simulink model "tb_q_current_control_basics"  (R2025b)
settings: Solver=VariableStepAuto  StartTime=0.0  StopTime=0.02  RelTol=1e-3
settings Model: Creator=semih  LastModifiedBy=semih

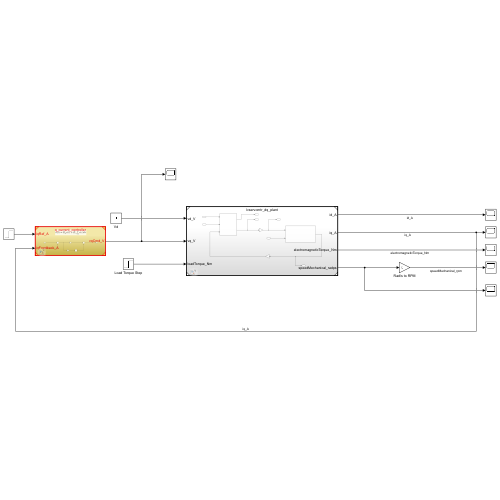
[thumbnail: Simulink's stored preview of the top-level diagram]
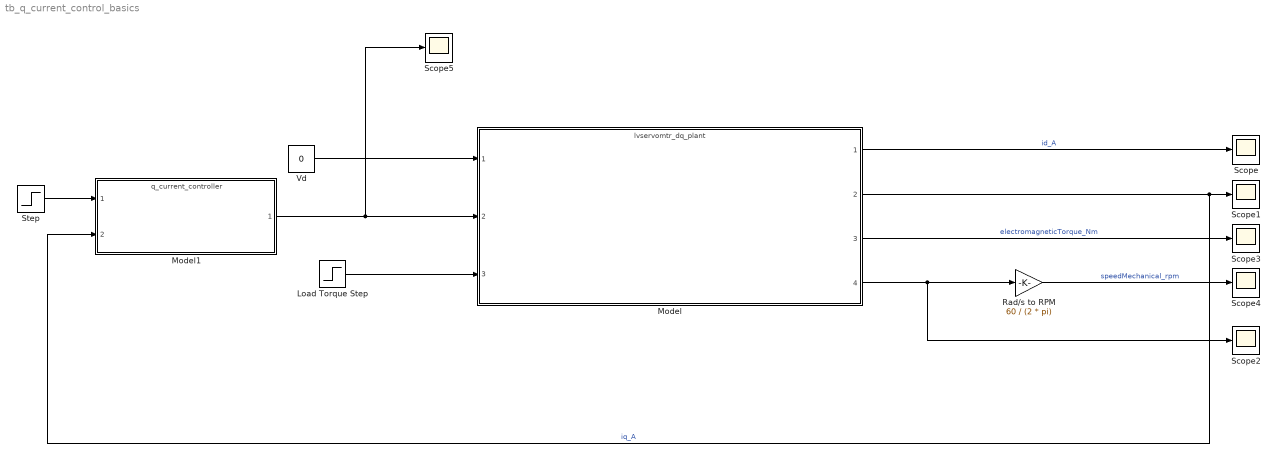
== system tb_q_current_control_basics ==
  Load Torque Step : Step  Time=0.030  After=0  SampleTime=0
  Model : ModelReference  ModelNameDialog=lvservomtr_dq_plant  SimulationMode=Normal  ModelReferenceVersion=1.7
  Model1 : ModelReference  ModelNameDialog=q_current_controller.slx  SimulationMode=Normal  ModelReferenceVersion=1.3
  Rad/s to RPM : Gain  Gain=60 / (2 * pi)
  Scope{,1..5} (6 alike) : Scope
      Scope settings: ActiveDisplayYMinimum=-0.42366511792142403  ActiveDisplayYMaximum=1.8876545573518515
      Scope1 settings: ActiveDisplayYMinimum=-0.63597233219420146  ActiveDisplayYMaximum=2.1211566623596005
      Scope2 settings: ActiveDisplayYMinimum=-14.648422716149396  ActiveDisplayYMaximum=131.83580444534459  DataLoggingVariableName=ScopeData2
      Scope3 settings: ActiveDisplayYMinimum=-0.077109095292808  ActiveDisplayYMaximum=0.69398185763527209  DataLoggingVariableName=ScopeData3
      Scope4 settings: ActiveDisplayYMinimum=-1818.6331248879962  ActiveDisplayYMaximum=1604.0491925649362  DataLoggingVariableName=ScopeData4
      Scope5 settings: ActiveDisplayYMinimum=-0.71634076865740015  ActiveDisplayYMaximum=3.1022847367350792  DataLoggingVariableName=ScopeData5
  Step : Step  Time=0.005  After=2  SampleTime=0
  Vd : Constant  Value=0
  wires:
  Load Torque Step/1 -> Model/3
  Rad/s to RPM/1 -> Scope4/1  "speedMechanical_rpm"
  Model/4 -> Scope2/1, Rad/s to RPM/1
  Model1/1 -> Scope5/1, Model/2
  Vd/1 -> Model/1
  Model/3 -> Scope3/1  "electromagneticTorque_Nm"
  Model/1 -> Scope/1  "id_A"
  Model/2 -> Model1/2, Scope1/1  "iq_A"
  Step/1 -> Model1/1
